simulink model "snap_adc5g_spec_rpi"  (R2019a)
settings: Solver=VariableStepDiscrete  StartTime=0.0  StopTime=10.0  RelTol=1e-3
undefined symbols (not defined in the file): pfb_coeff_gen_calc
libraries: xbsIndex_r4 x13965, casper_library_misc x80, casper_library_delays x43, xps_library x5, xbsReplacements_r4 x2, casper_library_communications x1
(part 133 of 152)

== system snap_adc5g_spec_rpi/fft_wideband_real/fft_biplex_real_4x/biplex_core/fft_stage_11/butterfly_direct/twiddle/bus_convert/conv3 ==
  note: (ones_bit & 1) -> round-to-even
      | (ones_bit ^ 1) -> round-to-odd
      | (sign_bit & 1)-> round-to-zero
      | (sign_bit ^ 1) -> round-to-inf
      | (X ~| 1) -> round half down
      | (X | 1) -> round half up
  in : Inport
  Concat : xbsIndex_r4/Concat  num_inputs=2  dbl_ovrd=off  block_type=concat
      settings: block_version=10.1.3
  Constant : xbsIndex_r4/Constant  const=1  gui_display_data_type=Fixed-point  arith_type=Unsigned  n_bits=1  bin_pt=0  preci_type=Single  exp_width=8  frac_width=24  explicit_period=off  period=1  equ=P=C  opselect=C  inp2=PCIN>>17  opr=+  inp1=P  carry=CIN  dbl_ovrd=off  block_type=constant
  Reinterpret : xbsIndex_r4/Reinterpret  force_arith_type=on  arith_type=Unsigned  force_bin_pt=on  bin_pt=0  block_type=reinterpret
      settings: infoedit="Changes signal type without altering the binary representation.   You can changed the signal between signed and unsigned, and relocate the binary point.<P><P>Hardware notes: In hardware this block costs nothing.<P><P>Example:  Suppose the input is 6 bits wide, signed, with 2 fractional bits, and the output is forced to unsigned with 0 fractional bits.  Then an input of -2.0 (1110.00 in binary 2's complement) becomes an output of 56 (111000 in binary)."  block_version=10.1.3
  adder : xbsIndex_r4/AddSub  mode=Addition  use_carryin=off  use_carryout=off  en=off  latency=1  precision=User Defined  arith_type="Signed  (2's comp)"  n_bits=19  bin_pt=17  quantization=Truncate  overflow=Wrap  use_behavioral_HDL=off  hw_selection=Fabric  pipelined=on  use_rpm=on  dbl_ovrd=off  block_type=addsub
      settings: xl_area=[0, 0, 0, 0, 0, 0, 0]  block_version=10.1.3
  almost_half : xbsIndex_r4/Constant  const=131071  gui_display_data_type=Fixed-point  arith_type=Unsigned  n_bits=35  bin_pt=0  preci_type=Single  exp_width=8  frac_width=24  explicit_period=off  period=1  equ=P=C  opselect=C  inp2=PCIN>>17  opr=+  inp1=P  carry=CIN  dbl_ovrd=off  block_type=constant
  bit : xbsIndex_r4/Slice  nbits=1  boolean_output=off  mode=Lower Bit Location + Width  bit1=0  base1=MSB of Input  bit0=17  base0=LSB of Input  dbl_ovrd=off  block_type=slice
      settings: infoedit="Extracts a given range of bits from each input sample and presents it at the output.  The output type is ordinarily unsigned with binary point at zero, but can be Boolean when the slice is one bit wide.<P><P>Hardware notes: In hardware this block costs nothing."  block_version=10.1.3
  force1 : xbsIndex_r4/Reinterpret  force_arith_type=on  arith_type="Signed  (2's comp)"  force_bin_pt=on  bin_pt=35  block_type=reinterpret
      settings: infoedit="Changes signal type without altering the binary representation.   You can changed the signal between signed and unsigned, and relocate the binary point.<P><P>Hardware notes: In hardware this block costs nothing.<P><P>Example:  Suppose the input is 6 bits wide, signed, with 2 fractional bits, and the output is forced to unsigned with 0 fractional bits.  Then an input of -2.0 (1110.00 in binary 2's complement) becomes an output of 56 (111000 in binary)."  block_version=10.1.3
  force2 : xbsIndex_r4/Reinterpret  force_arith_type=off  arith_type="Signed  (2's comp)"  force_bin_pt=on  bin_pt=35  block_type=reinterpret
      settings: infoedit="Changes signal type without altering the binary representation.   You can changed the signal between signed and unsigned, and relocate the binary point.<P><P>Hardware notes: In hardware this block costs nothing.<P><P>Example:  Suppose the input is 6 bits wide, signed, with 2 fractional bits, and the output is forced to unsigned with 0 fractional bits.  Then an input of -2.0 (1110.00 in binary 2's complement) becomes an output of 56 (111000 in binary)."  block_version=10.1.3
  tweak_op : xbsIndex_r4/Logical  logical_function=AND  inputs=2  en=off  latency=0  precision=Full  arith_type=Unsigned  n_bits=8  bin_pt=2  align_bp=on  dbl_ovrd=off  block_type=logical
      settings: xl_area=[0, 0, 0, 0, 0, 0, 0]
  out : Outport
  wires:
  tweak_op/1 -> Concat/2
  Constant/1 -> tweak_op/2
  bit/1 -> tweak_op/1
  almost_half/1 -> force2/1
  in/1 -> Reinterpret/1, bit/1
  Concat/1 -> force1/1
  Reinterpret/1 -> Concat/1
  force1/1 -> adder/1
  force2/1 -> adder/2
  adder/1 -> out/1

== system snap_adc5g_spec_rpi/fft_wideband_real/fft_biplex_real_4x/biplex_core/fft_stage_11/butterfly_direct/twiddle/bus_convert/conv4 ==
  note: (ones_bit & 1) -> round-to-even
      | (ones_bit ^ 1) -> round-to-odd
      | (sign_bit & 1)-> round-to-zero
      | (sign_bit ^ 1) -> round-to-inf
      | (X ~| 1) -> round half down
      | (X | 1) -> round half up
  in : Inport
  Concat : xbsIndex_r4/Concat  num_inputs=2  dbl_ovrd=off  block_type=concat
      settings: block_version=10.1.3
  Constant : xbsIndex_r4/Constant  const=1  gui_display_data_type=Fixed-point  arith_type=Unsigned  n_bits=1  bin_pt=0  preci_type=Single  exp_width=8  frac_width=24  explicit_period=off  period=1  equ=P=C  opselect=C  inp2=PCIN>>17  opr=+  inp1=P  carry=CIN  dbl_ovrd=off  block_type=constant
  Reinterpret : xbsIndex_r4/Reinterpret  force_arith_type=on  arith_type=Unsigned  force_bin_pt=on  bin_pt=0  block_type=reinterpret
      settings: infoedit="Changes signal type without altering the binary representation.   You can changed the signal between signed and unsigned, and relocate the binary point.<P><P>Hardware notes: In hardware this block costs nothing.<P><P>Example:  Suppose the input is 6 bits wide, signed, with 2 fractional bits, and the output is forced to unsigned with 0 fractional bits.  Then an input of -2.0 (1110.00 in binary 2's complement) becomes an output of 56 (111000 in binary)."  block_version=10.1.3
  adder : xbsIndex_r4/AddSub  mode=Addition  use_carryin=off  use_carryout=off  en=off  latency=1  precision=User Defined  arith_type="Signed  (2's comp)"  n_bits=19  bin_pt=17  quantization=Truncate  overflow=Wrap  use_behavioral_HDL=off  hw_selection=Fabric  pipelined=on  use_rpm=on  dbl_ovrd=off  block_type=addsub
      settings: xl_area=[0, 0, 0, 0, 0, 0, 0]  block_version=10.1.3
  almost_half : xbsIndex_r4/Constant  const=131071  gui_display_data_type=Fixed-point  arith_type=Unsigned  n_bits=35  bin_pt=0  preci_type=Single  exp_width=8  frac_width=24  explicit_period=off  period=1  equ=P=C  opselect=C  inp2=PCIN>>17  opr=+  inp1=P  carry=CIN  dbl_ovrd=off  block_type=constant
  bit : xbsIndex_r4/Slice  nbits=1  boolean_output=off  mode=Lower Bit Location + Width  bit1=0  base1=MSB of Input  bit0=17  base0=LSB of Input  dbl_ovrd=off  block_type=slice
      settings: infoedit="Extracts a given range of bits from each input sample and presents it at the output.  The output type is ordinarily unsigned with binary point at zero, but can be Boolean when the slice is one bit wide.<P><P>Hardware notes: In hardware this block costs nothing."  block_version=10.1.3
  force1 : xbsIndex_r4/Reinterpret  force_arith_type=on  arith_type="Signed  (2's comp)"  force_bin_pt=on  bin_pt=35  block_type=reinterpret
      settings: infoedit="Changes signal type without altering the binary representation.   You can changed the signal between signed and unsigned, and relocate the binary point.<P><P>Hardware notes: In hardware this block costs nothing.<P><P>Example:  Suppose the input is 6 bits wide, signed, with 2 fractional bits, and the output is forced to unsigned with 0 fractional bits.  Then an input of -2.0 (1110.00 in binary 2's complement) becomes an output of 56 (111000 in binary)."  block_version=10.1.3
  force2 : xbsIndex_r4/Reinterpret  force_arith_type=off  arith_type="Signed  (2's comp)"  force_bin_pt=on  bin_pt=35  block_type=reinterpret
      settings: infoedit="Changes signal type without altering the binary representation.   You can changed the signal between signed and unsigned, and relocate the binary point.<P><P>Hardware notes: In hardware this block costs nothing.<P><P>Example:  Suppose the input is 6 bits wide, signed, with 2 fractional bits, and the output is forced to unsigned with 0 fractional bits.  Then an input of -2.0 (1110.00 in binary 2's complement) becomes an output of 56 (111000 in binary)."  block_version=10.1.3
  tweak_op : xbsIndex_r4/Logical  logical_function=AND  inputs=2  en=off  latency=0  precision=Full  arith_type=Unsigned  n_bits=8  bin_pt=2  align_bp=on  dbl_ovrd=off  block_type=logical
      settings: xl_area=[0, 0, 0, 0, 0, 0, 0]
  out : Outport
  wires:
  tweak_op/1 -> Concat/2
  Constant/1 -> tweak_op/2
  bit/1 -> tweak_op/1
  almost_half/1 -> force2/1
  in/1 -> Reinterpret/1, bit/1
  Concat/1 -> force1/1
  Reinterpret/1 -> Concat/1
  force1/1 -> adder/1
  force2/1 -> adder/2
  adder/1 -> out/1

== system snap_adc5g_spec_rpi/fft_wideband_real/fft_biplex_real_4x/biplex_core/fft_stage_11/butterfly_direct/twiddle/bus_convert/debus ==
  bus_in : Inport
  reinterpret{1..4} (4 alike) : xbsIndex_r4/Reinterpret  force_arith_type=on  arith_type="Signed  (2's comp)"  force_bin_pt=on  bin_pt=34  block_type=reinterpret
  slice1 : xbsIndex_r4/Slice  nbits=37  boolean_output=off  mode=Upper Bit Location + Width  bit1=-111  base1=MSB of Input  bit0=0  base0=LSB of Input  dbl_ovrd=off  block_type=slice
  slice2 : xbsIndex_r4/Slice  nbits=37  boolean_output=off  mode=Upper Bit Location + Width  bit1=-74  base1=MSB of Input  bit0=0  base0=LSB of Input  dbl_ovrd=off  block_type=slice
  slice3 : xbsIndex_r4/Slice  nbits=37  boolean_output=off  mode=Upper Bit Location + Width  bit1=-37  base1=MSB of Input  bit0=0  base0=LSB of Input  dbl_ovrd=off  block_type=slice
  slice4 : xbsIndex_r4/Slice  nbits=37  boolean_output=off  mode=Upper Bit Location + Width  bit1=0  base1=MSB of Input  bit0=0  base0=LSB of Input  dbl_ovrd=off  block_type=slice
  msb_out4 : Outport
  out3 : Outport  Port=2
  out2 : Outport  Port=3
  lsb_out1 : Outport  Port=4
  wires:
  bus_in/1 -> slice4/1, slice3/1, slice2/1, slice1/1
  slice4/1 -> reinterpret4/1
  reinterpret4/1 -> msb_out4/1
  slice3/1 -> reinterpret3/1
  reinterpret3/1 -> out3/1
  slice2/1 -> reinterpret2/1
  reinterpret2/1 -> out2/1
  slice1/1 -> reinterpret1/1
  reinterpret1/1 -> lsb_out1/1

== system snap_adc5g_spec_rpi/fft_wideband_real/fft_biplex_real_4x/biplex_core/fft_stage_11/butterfly_direct/twiddle/bus_mult/a*b_bussify ==
  in1 : Inport
  in2 : Inport  Port=2
  concatenate : xbsIndex_r4/Concat  num_inputs=2  dbl_ovrd=off  block_type=concat
  reinterpret1 : xbsIndex_r4/Reinterpret  force_arith_type=on  arith_type=Unsigned  force_bin_pt=on  bin_pt=0  block_type=reinterpret
      settings: infoedit="Changes signal type without altering the binary representation.   You can changed the signal between signed and unsigned, and relocate the binary point.<br><br>Hardware notes: In hardware this block costs nothing.<br><br>Example:  Suppose the input is 6 bits wide, signed, with 2 fractional bits, and the output is forced to unsigned with 0 fractional bits.  Then an input of -2.0 (1110.00 in binary 2's complement) becomes an output of 56 (111000 in binary)."
  reinterpret2 : xbsIndex_r4/Reinterpret  force_arith_type=on  arith_type=Unsigned  force_bin_pt=on  bin_pt=0  block_type=reinterpret
      settings: infoedit="Changes signal type without altering the binary representation.   You can changed the signal between signed and unsigned, and relocate the binary point.<br><br>Hardware notes: In hardware this block costs nothing.<br><br>Example:  Suppose the input is 6 bits wide, signed, with 2 fractional bits, and the output is forced to unsigned with 0 fractional bits.  Then an input of -2.0 (1110.00 in binary 2's complement) becomes an output of 56 (111000 in binary)."
  bus_out : Outport
  wires:
  concatenate/1 -> bus_out/1
  in1/1 -> reinterpret1/1
  reinterpret1/1 -> concatenate/1
  in2/1 -> reinterpret2/1
  reinterpret2/1 -> concatenate/2

== system snap_adc5g_spec_rpi/fft_wideband_real/fft_biplex_real_4x/biplex_core/fft_stage_11/butterfly_direct/twiddle/bus_mult/a_debus ==
  bus_in : Inport
  reinterpret1 : xbsIndex_r4/Reinterpret  force_arith_type=on  arith_type=Unsigned  force_bin_pt=on  bin_pt=0  block_type=reinterpret
  slice1 : xbsIndex_r4/Slice  nbits=36  boolean_output=off  mode=Upper Bit Location + Width  bit1=0  base1=MSB of Input  bit0=0  base0=LSB of Input  dbl_ovrd=off  block_type=slice
  msb_lsb_out1 : Outport
  wires:
  bus_in/1 -> slice1/1
  slice1/1 -> reinterpret1/1
  reinterpret1/1 -> msb_lsb_out1/1

== system snap_adc5g_spec_rpi/fft_wideband_real/fft_biplex_real_4x/biplex_core/fft_stage_11/butterfly_direct/twiddle/bus_mult/b_debus ==
  bus_in : Inport
  reinterpret1 : xbsIndex_r4/Reinterpret  force_arith_type=on  arith_type=Unsigned  force_bin_pt=on  bin_pt=0  block_type=reinterpret
  reinterpret2 : xbsIndex_r4/Reinterpret  force_arith_type=on  arith_type=Unsigned  force_bin_pt=on  bin_pt=0  block_type=reinterpret
  slice1 : xbsIndex_r4/Slice  nbits=36  boolean_output=off  mode=Upper Bit Location + Width  bit1=-36  base1=MSB of Input  bit0=0  base0=LSB of Input  dbl_ovrd=off  block_type=slice
  slice2 : xbsIndex_r4/Slice  nbits=36  boolean_output=off  mode=Upper Bit Location + Width  bit1=0  base1=MSB of Input  bit0=0  base0=LSB of Input  dbl_ovrd=off  block_type=slice
  msb_out2 : Outport
  lsb_out1 : Outport  Port=2
  wires:
  bus_in/1 -> slice2/1, slice1/1
  slice2/1 -> reinterpret2/1
  reinterpret2/1 -> msb_out2/1
  slice1/1 -> reinterpret1/1
  reinterpret1/1 -> lsb_out1/1

== system snap_adc5g_spec_rpi/fft_wideband_real/fft_biplex_real_4x/biplex_core/fft_stage_11/butterfly_direct/twiddle/bus_mult/mult1 ==
  a : Inport
  b : Inport  Port=2
  a_expand : Subsystem  AncestorBlock=casper_library_flow_control/bus_expand  mask(bus_expand){mode=divisions of equal size, outputNum=4, outputWidth=[18 18 18 18], outputBinaryPt=[17 17 17 17], outputArithmeticType=[1 1 1 1], show_format=off, outputToWorkspace=off, variablePrefix=out, outputToModelAsWell=on}
      mask prompts: outputNum "Number of outputs:"; outputWidth "Output width:"; outputBinaryPt "Output binary point position:"; outputArithmeticType "Output arithmetic type (ufix=0, fix=1, bool=2):"; show_format "Print format string?"; outputToWorkspace "Output to workspace?"; variablePrefix "Variable name prefix:"; outputToModelAsWell "Output to model as well?"
      mask help:
      | Expands a 'bus' made using a bus_create or Xilinx
      | concat block.
      | The input will be divided into the specified number
      | of outputs with the specified arithmetic types.
      | Divisions are made from most significant bit.
      mask init: same as snap_adc5g_spec_rpi/ss_adc/ctrl_split
      settings: AttributesFormatString=4 outputs
      mask TypeOptions mode: divisions of equal size | divisions of arbitrary size
      mask Callback mode: bus_expand_callback();
      mask Callback outputWidth: bus_expand_callback();
      mask Callback outputToWorkspace: bus_expand_callback();
  a_replicate : Subsystem  AncestorBlock=casper_library_bus/bus_replicate  mask(bus_replicate){replication=2, csp_latency=1, misc=off, implementation=core}
      mask prompts: replication "replication factor"; csp_latency "latency"; misc "misc support"; implementation "delay implementation"
      mask help: Output bus formed by replicating input bus a number of times
      mask init:
      | bus_replicate_init(gcb, ...
      |     'replication', replication, ...
      |     'csp_latency', csp_latency, ...
      |     'implementation', implementation, ...
      |     'misc', misc);
      mask TypeOptions implementation: core | behavioral
  addsub_im : xbsIndex_r4/AddSub  mode=Addition  use_carryin=off  use_carryout=off  en=off  latency=1  precision=Full  arith_type=Unsigned  n_bits=16  bin_pt=14  quantization=Truncate  overflow=Wrap  use_behavioral_HDL=on  hw_selection=Fabric  pipelined=on  use_rpm=on  dbl_ovrd=off  block_type=addsub
  addsub_re : xbsIndex_r4/AddSub  mode=Subtraction  use_carryin=off  use_carryout=off  en=off  latency=1  precision=Full  arith_type=Unsigned  n_bits=16  bin_pt=14  quantization=Truncate  overflow=Wrap  use_behavioral_HDL=on  hw_selection=Fabric  pipelined=on  use_rpm=on  dbl_ovrd=off  block_type=addsub
  b_expand : Subsystem  AncestorBlock=casper_library_flow_control/bus_expand  mask(bus_expand){mode=divisions of equal size, outputNum=4, outputWidth=[18 18 18 18], outputBinaryPt=[17 17 17 17], outputArithmeticType=[1 1 1 1], show_format=off, outputToWorkspace=off, variablePrefix=out, outputToModelAsWell=on}
      mask prompts: outputNum "Number of outputs:"; outputWidth "Output width:"; outputBinaryPt "Output binary point position:"; outputArithmeticType "Output arithmetic type (ufix=0, fix=1, bool=2):"; show_format "Print format string?"; outputToWorkspace "Output to workspace?"; variablePrefix "Variable name prefix:"; outputToModelAsWell "Output to model as well?"
      mask help:
      | Expands a 'bus' made using a bus_create or Xilinx
      | concat block.
      | The input will be divided into the specified number
      | of outputs with the specified arithmetic types.
      | Divisions are made from most significant bit.
      mask init: same as snap_adc5g_spec_rpi/ss_adc/ctrl_split
      settings: AttributesFormatString=4 outputs
      mask TypeOptions mode: divisions of equal size | divisions of arbitrary size
      mask Callback mode: bus_expand_callback();
      mask Callback outputWidth: bus_expand_callback();
      mask Callback outputToWorkspace: bus_expand_callback();
  b_replicate : Subsystem  AncestorBlock=casper_library_bus/bus_replicate  mask(bus_replicate){replication=2, csp_latency=1, misc=off, implementation=core}
      mask prompts: replication "replication factor"; csp_latency "latency"; misc "misc support"; implementation "delay implementation"
      mask help: Output bus formed by replicating input bus a number of times
      mask init:
      | bus_replicate_init(gcb, ...
      |     'replication', replication, ...
      |     'csp_latency', csp_latency, ...
      |     'implementation', implementation, ...
      |     'misc', misc);
      mask TypeOptions implementation: core | behavioral
  convert_im : xbsIndex_r4/Convert  gui_display_data_type=Fixed-point  arith_type="Signed  (2's comp)"  n_bits=37  bin_pt=34  float_type=Single  exp_bits=8  fraction_bits=24  quantization=Truncate  overflow=Wrap  en=off  latency=0  pipeline=on  dbl_ovrd=off  block_type=convert
  convert_re : xbsIndex_r4/Convert  gui_display_data_type=Fixed-point  arith_type="Signed  (2's comp)"  n_bits=37  bin_pt=34  float_type=Single  exp_bits=8  fraction_bits=24  quantization=Truncate  overflow=Wrap  en=off  latency=0  pipeline=on  dbl_ovrd=off  block_type=convert
  imim : xbsIndex_r4/Mult  precision=Full  arith_type="Signed  (2's comp)"  n_bits=16  bin_pt=14  quantization=Truncate  overflow=Wrap  en=off  latency=2  use_behavioral_HDL=on  opt=Speed  use_embedded=off  optimum_pipeline=off  pipeline=on  dbl_ovrd=off  use_rpm=on  placement_style=Triangular  block_type=mult
  imre : xbsIndex_r4/Mult  precision=Full  arith_type="Signed  (2's comp)"  n_bits=16  bin_pt=14  quantization=Truncate  overflow=Wrap  en=off  latency=2  use_behavioral_HDL=on  opt=Speed  use_embedded=off  optimum_pipeline=off  pipeline=on  dbl_ovrd=off  use_rpm=on  placement_style=Triangular  block_type=mult
  reim : xbsIndex_r4/Mult  precision=Full  arith_type="Signed  (2's comp)"  n_bits=16  bin_pt=14  quantization=Truncate  overflow=Wrap  en=off  latency=2  use_behavioral_HDL=on  opt=Speed  use_embedded=off  optimum_pipeline=off  pipeline=on  dbl_ovrd=off  use_rpm=on  placement_style=Triangular  block_type=mult
  rere : xbsIndex_r4/Mult  precision=Full  arith_type="Signed  (2's comp)"  n_bits=16  bin_pt=14  quantization=Truncate  overflow=Wrap  en=off  latency=2  use_behavioral_HDL=on  opt=Speed  use_embedded=off  optimum_pipeline=off  pipeline=on  dbl_ovrd=off  use_rpm=on  placement_style=Triangular  block_type=mult
  ri_to_c : Subsystem  AncestorBlock=casper_library_misc/ri_to_c  mask(ri_to_c){}
      mask help:
      | Concatenates real and imaginary inputs into a complex output.
      | Useful for simplifying interconnects.
      | See also: Complex to Real-Imag (c_to_ri)
      mask Help: eval('xlWeb(''http://casper.berkeley.edu/wiki/Ri_to_c'')')
  ab : Outport
  wires:
  a/1 -> a_replicate/1(in)
  b/1 -> b_replicate/1(in)
  a_replicate/1(out) -> a_expand/1(bus_in)
  b_replicate/1(out) -> b_expand/1(bus_in)
  a_expand/1(msb_out4) -> rere/1
  b_expand/1(msb_out4) -> rere/2
  a_expand/2(out3) -> imim/1
  b_expand/2(out3) -> imim/2
  a_expand/4(lsb_out1) -> imre/1
  b_expand/3(out2) -> imre/2
  a_expand/3(out2) -> reim/1
  b_expand/4(lsb_out1) -> reim/2
  rere/1 -> addsub_re/1
  imim/1 -> addsub_re/2
  imre/1 -> addsub_im/1
  reim/1 -> addsub_im/2
  addsub_re/1 -> convert_re/1
  addsub_im/1 -> convert_im/1
  convert_re/1 -> ri_to_c/1(re)
  convert_im/1 -> ri_to_c/2(im)
  ri_to_c/1(c) -> ab/1

== system snap_adc5g_spec_rpi/fft_wideband_real/fft_biplex_real_4x/biplex_core/fft_stage_11/butterfly_direct/twiddle/bus_mult/mult2 ==
  a : Inport
  b : Inport  Port=2
  a_expand : Subsystem  AncestorBlock=casper_library_flow_control/bus_expand  mask(bus_expand){mode=divisions of equal size, outputNum=4, outputWidth=[18 18 18 18], outputBinaryPt=[17 17 17 17], outputArithmeticType=[1 1 1 1], show_format=off, outputToWorkspace=off, variablePrefix=out, outputToModelAsWell=on}
      mask prompts: outputNum "Number of outputs:"; outputWidth "Output width:"; outputBinaryPt "Output binary point position:"; outputArithmeticType "Output arithmetic type (ufix=0, fix=1, bool=2):"; show_format "Print format string?"; outputToWorkspace "Output to workspace?"; variablePrefix "Variable name prefix:"; outputToModelAsWell "Output to model as well?"
      mask help:
      | Expands a 'bus' made using a bus_create or Xilinx
      | concat block.
      | The input will be divided into the specified number
      | of outputs with the specified arithmetic types.
      | Divisions are made from most significant bit.
      mask init: same as snap_adc5g_spec_rpi/ss_adc/ctrl_split
      settings: AttributesFormatString=4 outputs
      mask TypeOptions mode: divisions of equal size | divisions of arbitrary size
      mask Callback mode: bus_expand_callback();
      mask Callback outputWidth: bus_expand_callback();
      mask Callback outputToWorkspace: bus_expand_callback();
  a_replicate : Subsystem  AncestorBlock=casper_library_bus/bus_replicate  mask(bus_replicate){replication=2, csp_latency=1, misc=off, implementation=core}
      mask prompts: replication "replication factor"; csp_latency "latency"; misc "misc support"; implementation "delay implementation"
      mask help: Output bus formed by replicating input bus a number of times
      mask init:
      | bus_replicate_init(gcb, ...
      |     'replication', replication, ...
      |     'csp_latency', csp_latency, ...
      |     'implementation', implementation, ...
      |     'misc', misc);
      mask TypeOptions implementation: core | behavioral
  addsub_im : xbsIndex_r4/AddSub  mode=Addition  use_carryin=off  use_carryout=off  en=off  latency=1  precision=Full  arith_type=Unsigned  n_bits=16  bin_pt=14  quantization=Truncate  overflow=Wrap  use_behavioral_HDL=on  hw_selection=Fabric  pipelined=on  use_rpm=on  dbl_ovrd=off  block_type=addsub
  addsub_re : xbsIndex_r4/AddSub  mode=Subtraction  use_carryin=off  use_carryout=off  en=off  latency=1  precision=Full  arith_type=Unsigned  n_bits=16  bin_pt=14  quantization=Truncate  overflow=Wrap  use_behavioral_HDL=on  hw_selection=Fabric  pipelined=on  use_rpm=on  dbl_ovrd=off  block_type=addsub
  b_expand : Subsystem  AncestorBlock=casper_library_flow_control/bus_expand  mask(bus_expand){mode=divisions of equal size, outputNum=4, outputWidth=[18 18 18 18], outputBinaryPt=[17 17 17 17], outputArithmeticType=[1 1 1 1], show_format=off, outputToWorkspace=off, variablePrefix=out, outputToModelAsWell=on}
      mask prompts: outputNum "Number of outputs:"; outputWidth "Output width:"; outputBinaryPt "Output binary point position:"; outputArithmeticType "Output arithmetic type (ufix=0, fix=1, bool=2):"; show_format "Print format string?"; outputToWorkspace "Output to workspace?"; variablePrefix "Variable name prefix:"; outputToModelAsWell "Output to model as well?"
      mask help:
      | Expands a 'bus' made using a bus_create or Xilinx
      | concat block.
      | The input will be divided into the specified number
      | of outputs with the specified arithmetic types.
      | Divisions are made from most significant bit.
      mask init: same as snap_adc5g_spec_rpi/ss_adc/ctrl_split
      settings: AttributesFormatString=4 outputs
      mask TypeOptions mode: divisions of equal size | divisions of arbitrary size
      mask Callback mode: bus_expand_callback();
      mask Callback outputWidth: bus_expand_callback();
      mask Callback outputToWorkspace: bus_expand_callback();
  b_replicate : Subsystem  AncestorBlock=casper_library_bus/bus_replicate  mask(bus_replicate){replication=2, csp_latency=1, misc=off, implementation=core}
      mask prompts: replication "replication factor"; csp_latency "latency"; misc "misc support"; implementation "delay implementation"
      mask help: Output bus formed by replicating input bus a number of times
      mask init:
      | bus_replicate_init(gcb, ...
      |     'replication', replication, ...
      |     'csp_latency', csp_latency, ...
      |     'implementation', implementation, ...
      |     'misc', misc);
      mask TypeOptions implementation: core | behavioral
  convert_im : xbsIndex_r4/Convert  gui_display_data_type=Fixed-point  arith_type="Signed  (2's comp)"  n_bits=37  bin_pt=34  float_type=Single  exp_bits=8  fraction_bits=24  quantization=Truncate  overflow=Wrap  en=off  latency=0  pipeline=on  dbl_ovrd=off  block_type=convert
  convert_re : xbsIndex_r4/Convert  gui_display_data_type=Fixed-point  arith_type="Signed  (2's comp)"  n_bits=37  bin_pt=34  float_type=Single  exp_bits=8  fraction_bits=24  quantization=Truncate  overflow=Wrap  en=off  latency=0  pipeline=on  dbl_ovrd=off  block_type=convert
  imim : xbsIndex_r4/Mult  precision=Full  arith_type="Signed  (2's comp)"  n_bits=16  bin_pt=14  quantization=Truncate  overflow=Wrap  en=off  latency=2  use_behavioral_HDL=on  opt=Speed  use_embedded=off  optimum_pipeline=off  pipeline=on  dbl_ovrd=off  use_rpm=on  placement_style=Triangular  block_type=mult
  imre : xbsIndex_r4/Mult  precision=Full  arith_type="Signed  (2's comp)"  n_bits=16  bin_pt=14  quantization=Truncate  overflow=Wrap  en=off  latency=2  use_behavioral_HDL=on  opt=Speed  use_embedded=off  optimum_pipeline=off  pipeline=on  dbl_ovrd=off  use_rpm=on  placement_style=Triangular  block_type=mult
  reim : xbsIndex_r4/Mult  precision=Full  arith_type="Signed  (2's comp)"  n_bits=16  bin_pt=14  quantization=Truncate  overflow=Wrap  en=off  latency=2  use_behavioral_HDL=on  opt=Speed  use_embedded=off  optimum_pipeline=off  pipeline=on  dbl_ovrd=off  use_rpm=on  placement_style=Triangular  block_type=mult
  rere : xbsIndex_r4/Mult  precision=Full  arith_type="Signed  (2's comp)"  n_bits=16  bin_pt=14  quantization=Truncate  overflow=Wrap  en=off  latency=2  use_behavioral_HDL=on  opt=Speed  use_embedded=off  optimum_pipeline=off  pipeline=on  dbl_ovrd=off  use_rpm=on  placement_style=Triangular  block_type=mult
  ri_to_c : Subsystem  AncestorBlock=casper_library_misc/ri_to_c  mask(ri_to_c){}
      mask help:
      | Concatenates real and imaginary inputs into a complex output.
      | Useful for simplifying interconnects.
      | See also: Complex to Real-Imag (c_to_ri)
      mask Help: eval('xlWeb(''http://casper.berkeley.edu/wiki/Ri_to_c'')')
  ab : Outport
  wires:
  a/1 -> a_replicate/1(in)
  b/1 -> b_replicate/1(in)
  a_replicate/1(out) -> a_expand/1(bus_in)
  b_replicate/1(out) -> b_expand/1(bus_in)
  a_expand/1(msb_out4) -> rere/1
  b_expand/1(msb_out4) -> rere/2
  a_expand/2(out3) -> imim/1
  b_expand/2(out3) -> imim/2
  a_expand/4(lsb_out1) -> imre/1
  b_expand/3(out2) -> imre/2
  a_expand/3(out2) -> reim/1
  b_expand/4(lsb_out1) -> reim/2
  rere/1 -> addsub_re/1
  imim/1 -> addsub_re/2
  imre/1 -> addsub_im/1
  reim/1 -> addsub_im/2
  addsub_re/1 -> convert_re/1
  addsub_im/1 -> convert_im/1
  convert_re/1 -> ri_to_c/1(re)
  convert_im/1 -> ri_to_c/2(im)
  ri_to_c/1(c) -> ab/1

== system snap_adc5g_spec_rpi/fft_wideband_real/fft_biplex_real_4x/biplex_core/fft_stage_11/butterfly_direct/twiddle/bus_mult/repa ==
  in : Inport
  bussify : Subsystem  AncestorBlock=casper_library_flow_control/bus_create  mask(bus_create){inputNum=1}
      mask prompts: inputNum "Number of inputs:"
      mask init:
      | bus_create_init(gcb,...
      |     'inputNum', inputNum);
  din0_0 : xbsIndex_r4/Delay  rst=off  infoeditControl=Selection of Reset will increase slice count due to use of real FFs and instead of SRLs  en=off  latency=1  reg_retiming=off  dbl_ovrd=off  block_type=delay
  out : Outport
  wires:
  in/1 -> din0_0/1
  din0_0/1 -> bussify/1(in1)
  bussify/1(bus_out) -> out/1

== system snap_adc5g_spec_rpi/fft_wideband_real/fft_biplex_real_4x/biplex_core/fft_stage_11/butterfly_direct/twiddle/bus_mult/repb ==
  in : Inport
  bussify : Subsystem  AncestorBlock=casper_library_flow_control/bus_create  mask(bus_create){inputNum=1}
      mask prompts: inputNum "Number of inputs:"
      mask init:
      | bus_create_init(gcb,...
      |     'inputNum', inputNum);
  din0_0 : xbsIndex_r4/Delay  rst=off  infoeditControl=Selection of Reset will increase slice count due to use of real FFs and instead of SRLs  en=off  latency=1  reg_retiming=off  dbl_ovrd=off  block_type=delay
  out : Outport
  wires:
  in/1 -> din0_0/1
  din0_0/1 -> bussify/1(in1)
  bussify/1(bus_out) -> out/1

== system snap_adc5g_spec_rpi/fft_wideband_real/fft_biplex_real_4x/biplex_core/fft_stage_11/butterfly_direct/twiddle/coeff_gen/bit_reverse ==
  in : Inport
  bit0 : xbsIndex_r4/Slice  nbits=1  boolean_output=off  mode=Lower Bit Location + Width  bit1=0  base1=MSB of Input  bit0=0  base0=LSB of Input  dbl_ovrd=off  block_type=slice
  bit1 : xbsIndex_r4/Slice  nbits=1  boolean_output=off  mode=Lower Bit Location + Width  bit1=0  base1=MSB of Input  bit0=1  base0=LSB of Input  dbl_ovrd=off  block_type=slice
  bit2 : xbsIndex_r4/Slice  nbits=1  boolean_output=off  mode=Lower Bit Location + Width  bit1=0  base1=MSB of Input  bit0=2  base0=LSB of Input  dbl_ovrd=off  block_type=slice
  bit3 : xbsIndex_r4/Slice  nbits=1  boolean_output=off  mode=Lower Bit Location + Width  bit1=0  base1=MSB of Input  bit0=3  base0=LSB of Input  dbl_ovrd=off  block_type=slice
  bit4 : xbsIndex_r4/Slice  nbits=1  boolean_output=off  mode=Lower Bit Location + Width  bit1=0  base1=MSB of Input  bit0=4  base0=LSB of Input  dbl_ovrd=off  block_type=slice
  bit5 : xbsIndex_r4/Slice  nbits=1  boolean_output=off  mode=Lower Bit Location + Width  bit1=0  base1=MSB of Input  bit0=5  base0=LSB of Input  dbl_ovrd=off  block_type=slice
  bit6 : xbsIndex_r4/Slice  nbits=1  boolean_output=off  mode=Lower Bit Location + Width  bit1=0  base1=MSB of Input  bit0=6  base0=LSB of Input  dbl_ovrd=off  block_type=slice
  bit7 : xbsIndex_r4/Slice  nbits=1  boolean_output=off  mode=Lower Bit Location + Width  bit1=0  base1=MSB of Input  bit0=7  base0=LSB of Input  dbl_ovrd=off  block_type=slice
  bit8 : xbsIndex_r4/Slice  nbits=1  boolean_output=off  mode=Lower Bit Location + Width  bit1=0  base1=MSB of Input  bit0=8  base0=LSB of Input  dbl_ovrd=off  block_type=slice
  bit9 : xbsIndex_r4/Slice  nbits=1  boolean_output=off  mode=Lower Bit Location + Width  bit1=0  base1=MSB of Input  bit0=9  base0=LSB of Input  dbl_ovrd=off  block_type=slice
  concat : xbsIndex_r4/Concat  num_inputs=10  dbl_ovrd=off  block_type=concat
  out : Outport
  wires:
  in/1 -> bit9/1, bit8/1, bit7/1, bit6/1, bit5/1, bit4/1, bit3/1, bit2/1, bit1/1, bit0/1
  bit9/1 -> concat/10
  bit8/1 -> concat/9
  bit7/1 -> concat/8
  bit6/1 -> concat/7
  bit5/1 -> concat/6
  bit4/1 -> concat/5
  bit3/1 -> concat/4
  bit2/1 -> concat/3
  bit1/1 -> concat/2
  bit0/1 -> concat/1
  concat/1 -> out/1

== system snap_adc5g_spec_rpi/fft_wideband_real/fft_biplex_real_4x/biplex_core/fft_stage_11/butterfly_direct/twiddle/coeff_gen/cosin ==
  theta : Inport
  misci : Inport  Port=2
  Constant : xbsIndex_r4/Constant  const=0  gui_display_data_type=Fixed-point  arith_type=Signed (2's comp)  n_bits=n_bits  bin_pt=bin_pt  preci_type=Single  exp_width=8  frac_width=24  explicit_period=off  period=1  equ=P=C  opselect=C  inp2=PCIN>>17  opr=+  inp1=P  carry=CIN  dbl_ovrd=off  block_type=constant
  Constant1 : xbsIndex_r4/Constant  const=0  gui_display_data_type=Fixed-point  arith_type=Signed (2's comp)  n_bits=n_bits  bin_pt=bin_pt  preci_type=Single  exp_width=8  frac_width=24  explicit_period=off  period=1  equ=P=C  opselect=C  inp2=PCIN>>17  opr=+  inp1=P  carry=CIN  dbl_ovrd=off  block_type=constant
  Constant2 : xbsIndex_r4/Constant  const=0  gui_display_data_type=Fixed-point  arith_type=Boolean  n_bits=n_bits  bin_pt=bin_pt  preci_type=Single  exp_width=8  frac_width=24  explicit_period=off  period=1  equ=P=C  opselect=C  inp2=PCIN>>17  opr=+  inp1=P  carry=CIN  dbl_ovrd=off  block_type=constant
  Constant3 : xbsIndex_r4/Constant  const=0  gui_display_data_type=Fixed-point  arith_type=Boolean  n_bits=n_bits  bin_pt=bin_pt  preci_type=Single  exp_width=8  frac_width=24  explicit_period=off  period=1  equ=P=C  opselect=C  inp2=PCIN>>17  opr=+  inp1=P  carry=CIN  dbl_ovrd=off  block_type=constant
  Constant4 : xbsIndex_r4/Constant  const=0  gui_display_data_type=Fixed-point  arith_type=Unsigned  n_bits=1  bin_pt=0  preci_type=Single  exp_width=8  frac_width=24  explicit_period=on  period=1  equ=P=C  opselect=C  inp2=PCIN>>17  opr=+  inp1=P  carry=CIN  dbl_ovrd=off  block_type=constant
  Constant5 : xbsIndex_r4/Constant  const=0  gui_display_data_type=Fixed-point  arith_type=Unsigned  n_bits=1  bin_pt=0  preci_type=Single  exp_width=8  frac_width=24  explicit_period=on  period=1  equ=P=C  opselect=C  inp2=PCIN>>17  opr=+  inp1=P  carry=CIN  dbl_ovrd=off  block_type=constant
  Delay : xbsIndex_r4/Delay  rst=off  infoeditControl=Selection of Reset will increase slice count due to use of real FFs and instead of SRLs  en=off  latency=bram_latency  reg_retiming=on  dbl_ovrd=off  block_type=delay
  Delay10 : xbsIndex_r4/Delay  rst=off  infoeditControl=Selection of Reset will increase slice count due to use of real FFs and instead of SRLs  en=off  latency=bram_latency  reg_retiming=on  dbl_ovrd=off  block_type=delay
  Delay8 : xbsIndex_r4/Delay  rst=off  infoeditControl=Selection of Reset will increase slice count due to use of real FFs and instead of SRLs  en=off  latency=bram_latency  reg_retiming=on  dbl_ovrd=off  block_type=delay
  Terminator : Terminator
  Terminator1 : Terminator
  add_convert0 : Subsystem
  add_convert1 : Subsystem
  assert : xbsIndex_r4/Assert  assert_type=on  type_source=Explicitly  gui_display_data_type=Fixed-point  arith_type=Unsigned  n_bits=10  bin_pt=0  preci_type=Single  exp_width=8  frac_width=24  assert_rate=off  rate_source=Explicitly  period=1  output_port=on  block_type=assert
  invert0 : Subsystem  mask{n_bits=n_bits, bin_pt=bin_pt, neg_latency=neg_latency, mux_latency=mux_latency}
      mask prompts: n_bits "bit width"; bin_pt "binary point"; neg_latency "negate latency"; mux_latency "mux latency"
  invert1 : Subsystem  mask{n_bits=n_bits, bin_pt=bin_pt, neg_latency=neg_latency, mux_latency=mux_latency}
      mask prompts: n_bits "bit width"; bin_pt "binary point"; neg_latency "negate latency"; mux_latency "mux latency"
  lookup : xbsIndex_r4/Dual Port RAM  depth=2^(10)  initVector=cos((0*(2*pi))+(2*pi)/(2^11)*(0:(2^10)-1))  distributed_mem=Block RAM  init_a=0  init_b=0  rst_a=off  rst_b=off  en_a=off  en_b=off  latency=bram_latency  write_mode_A=Read After Write  write_mode_B=Read After Write  optimize=Area  dbl_ovrd=off  block_type=dpram
  cos : Outport
  -sin : Outport  Port=2
  misco : Outport  Port=3
  wires:
  theta/1 -> assert/1
  assert/1 -> add_convert0/1(theta), add_convert1/1(theta)
  Constant4/1 -> add_convert0/2(misci)
  add_convert0/3(misco) -> Terminator/1
  misci/1 -> add_convert1/2(misci)
  add_convert1/3(misco) -> Delay/1
  add_convert0/2(add) -> lookup/1
  add_convert1/2(add) -> lookup/4
  Constant/1 -> lookup/2
  Constant2/1 -> lookup/3
  Constant1/1 -> lookup/5
  Constant3/1 -> lookup/6
  add_convert1/1(negate) -> Delay8/1
  add_convert0/1(negate) -> Delay10/1
  Delay10/1 -> invert0/1(negate)
  Constant5/1 -> invert0/3(misci)
  lookup/1 -> invert0/2(in)
  Delay8/1 -> invert1/1(negate)
  lookup/2 -> invert1/2(in)
  invert0/2(misco) -> Terminator1/1
  Delay/1 -> invert1/3(misci)
  invert0/1(out) -> cos/1
  invert1/1(out) -> -sin/1
  invert1/2(misco) -> misco/1

== system snap_adc5g_spec_rpi/fft_wideband_real/fft_biplex_real_4x/biplex_core/fft_stage_2/butterfly_direct/bus_convert/conv1/convert ==
  note: (ones_bit & 1) -> round-to-even
      | (ones_bit ^ 1) -> round-to-odd
      | (sign_bit & 1)-> round-to-zero
      | (sign_bit ^ 1) -> round-to-inf
      | (X ~| 1) -> round half down
      | (X | 1) -> round half up
  in : Inport
  Concat : xbsIndex_r4/Concat  num_inputs=2  dbl_ovrd=off  block_type=concat
      settings: block_version=10.1.3
  Constant : xbsIndex_r4/Constant  const=1  gui_display_data_type=Fixed-point  arith_type=Unsigned  n_bits=1  bin_pt=0  preci_type=Single  exp_width=8  frac_width=24  explicit_period=off  period=1  equ=P=C  opselect=C  inp2=PCIN>>17  opr=+  inp1=P  carry=CIN  dbl_ovrd=off  block_type=constant
  Reinterpret : xbsIndex_r4/Reinterpret  force_arith_type=on  arith_type=Unsigned  force_bin_pt=on  bin_pt=0  block_type=reinterpret
      settings: infoedit="Changes signal type without altering the binary representation.   You can changed the signal between signed and unsigned, and relocate the binary point.<P><P>Hardware notes: In hardware this block costs nothing.<P><P>Example:  Suppose the input is 6 bits wide, signed, with 2 fractional bits, and the output is forced to unsigned with 0 fractional bits.  Then an input of -2.0 (1110.00 in binary 2's complement) becomes an output of 56 (111000 in binary)."  block_version=10.1.3
  adder : xbsIndex_r4/AddSub  mode=Addition  use_carryin=off  use_carryout=off  en=off  latency=1  precision=User Defined  arith_type="Signed  (2's comp)"  n_bits=18  bin_pt=17  quantization=Truncate  overflow=Wrap  use_behavioral_HDL=off  hw_selection=Fabric  pipelined=on  use_rpm=on  dbl_ovrd=off  block_type=addsub
      settings: xl_area=[0, 0, 0, 0, 0, 0, 0]  block_version=10.1.3
  almost_half : xbsIndex_r4/Constant  const=1  gui_display_data_type=Fixed-point  arith_type=Unsigned  n_bits=19  bin_pt=0  preci_type=Single  exp_width=8  frac_width=24  explicit_period=off  period=1  equ=P=C  opselect=C  inp2=PCIN>>17  opr=+  inp1=P  carry=CIN  dbl_ovrd=off  block_type=constant
  bit : xbsIndex_r4/Slice  nbits=1  boolean_output=off  mode=Lower Bit Location + Width  bit1=0  base1=MSB of Input  bit0=1  base0=LSB of Input  dbl_ovrd=off  block_type=slice
      settings: infoedit="Extracts a given range of bits from each input sample and presents it at the output.  The output type is ordinarily unsigned with binary point at zero, but can be Boolean when the slice is one bit wide.<P><P>Hardware notes: In hardware this block costs nothing."  block_version=10.1.3
  force1 : xbsIndex_r4/Reinterpret  force_arith_type=on  arith_type="Signed  (2's comp)"  force_bin_pt=on  bin_pt=19  block_type=reinterpret
      settings: infoedit="Changes signal type without altering the binary representation.   You can changed the signal between signed and unsigned, and relocate the binary point.<P><P>Hardware notes: In hardware this block costs nothing.<P><P>Example:  Suppose the input is 6 bits wide, signed, with 2 fractional bits, and the output is forced to unsigned with 0 fractional bits.  Then an input of -2.0 (1110.00 in binary 2's complement) becomes an output of 56 (111000 in binary)."  block_version=10.1.3
  force2 : xbsIndex_r4/Reinterpret  force_arith_type=off  arith_type="Signed  (2's comp)"  force_bin_pt=on  bin_pt=19  block_type=reinterpret
      settings: infoedit="Changes signal type without altering the binary representation.   You can changed the signal between signed and unsigned, and relocate the binary point.<P><P>Hardware notes: In hardware this block costs nothing.<P><P>Example:  Suppose the input is 6 bits wide, signed, with 2 fractional bits, and the output is forced to unsigned with 0 fractional bits.  Then an input of -2.0 (1110.00 in binary 2's complement) becomes an output of 56 (111000 in binary)."  block_version=10.1.3
  tweak_op : xbsIndex_r4/Logical  logical_function=AND  inputs=2  en=off  latency=0  precision=Full  arith_type=Unsigned  n_bits=8  bin_pt=2  align_bp=on  dbl_ovrd=off  block_type=logical
      settings: xl_area=[0, 0, 0, 0, 0, 0, 0]
  out : Outport
  wires:
  tweak_op/1 -> Concat/2
  Constant/1 -> tweak_op/2
  bit/1 -> tweak_op/1
  almost_half/1 -> force2/1
  in/1 -> Reinterpret/1, bit/1
  Concat/1 -> force1/1
  Reinterpret/1 -> Concat/1
  force1/1 -> adder/1
  force2/1 -> adder/2
  adder/1 -> out/1

== system snap_adc5g_spec_rpi/fft_wideband_real/fft_biplex_real_4x/biplex_core/fft_stage_2/butterfly_direct/bus_convert/conv2/convert ==
  note: (ones_bit & 1) -> round-to-even
      | (ones_bit ^ 1) -> round-to-odd
      | (sign_bit & 1)-> round-to-zero
      | (sign_bit ^ 1) -> round-to-inf
      | (X ~| 1) -> round half down
      | (X | 1) -> round half up
  in : Inport
  Concat : xbsIndex_r4/Concat  num_inputs=2  dbl_ovrd=off  block_type=concat
      settings: block_version=10.1.3
  Constant : xbsIndex_r4/Constant  const=1  gui_display_data_type=Fixed-point  arith_type=Unsigned  n_bits=1  bin_pt=0  preci_type=Single  exp_width=8  frac_width=24  explicit_period=off  period=1  equ=P=C  opselect=C  inp2=PCIN>>17  opr=+  inp1=P  carry=CIN  dbl_ovrd=off  block_type=constant
  Reinterpret : xbsIndex_r4/Reinterpret  force_arith_type=on  arith_type=Unsigned  force_bin_pt=on  bin_pt=0  block_type=reinterpret
      settings: infoedit="Changes signal type without altering the binary representation.   You can changed the signal between signed and unsigned, and relocate the binary point.<P><P>Hardware notes: In hardware this block costs nothing.<P><P>Example:  Suppose the input is 6 bits wide, signed, with 2 fractional bits, and the output is forced to unsigned with 0 fractional bits.  Then an input of -2.0 (1110.00 in binary 2's complement) becomes an output of 56 (111000 in binary)."  block_version=10.1.3
  adder : xbsIndex_r4/AddSub  mode=Addition  use_carryin=off  use_carryout=off  en=off  latency=1  precision=User Defined  arith_type="Signed  (2's comp)"  n_bits=18  bin_pt=17  quantization=Truncate  overflow=Wrap  use_behavioral_HDL=off  hw_selection=Fabric  pipelined=on  use_rpm=on  dbl_ovrd=off  block_type=addsub
      settings: xl_area=[0, 0, 0, 0, 0, 0, 0]  block_version=10.1.3
  almost_half : xbsIndex_r4/Constant  const=1  gui_display_data_type=Fixed-point  arith_type=Unsigned  n_bits=19  bin_pt=0  preci_type=Single  exp_width=8  frac_width=24  explicit_period=off  period=1  equ=P=C  opselect=C  inp2=PCIN>>17  opr=+  inp1=P  carry=CIN  dbl_ovrd=off  block_type=constant
  bit : xbsIndex_r4/Slice  nbits=1  boolean_output=off  mode=Lower Bit Location + Width  bit1=0  base1=MSB of Input  bit0=1  base0=LSB of Input  dbl_ovrd=off  block_type=slice
      settings: infoedit="Extracts a given range of bits from each input sample and presents it at the output.  The output type is ordinarily unsigned with binary point at zero, but can be Boolean when the slice is one bit wide.<P><P>Hardware notes: In hardware this block costs nothing."  block_version=10.1.3
  force1 : xbsIndex_r4/Reinterpret  force_arith_type=on  arith_type="Signed  (2's comp)"  force_bin_pt=on  bin_pt=19  block_type=reinterpret
      settings: infoedit="Changes signal type without altering the binary representation.   You can changed the signal between signed and unsigned, and relocate the binary point.<P><P>Hardware notes: In hardware this block costs nothing.<P><P>Example:  Suppose the input is 6 bits wide, signed, with 2 fractional bits, and the output is forced to unsigned with 0 fractional bits.  Then an input of -2.0 (1110.00 in binary 2's complement) becomes an output of 56 (111000 in binary)."  block_version=10.1.3
  force2 : xbsIndex_r4/Reinterpret  force_arith_type=off  arith_type="Signed  (2's comp)"  force_bin_pt=on  bin_pt=19  block_type=reinterpret
      settings: infoedit="Changes signal type without altering the binary representation.   You can changed the signal between signed and unsigned, and relocate the binary point.<P><P>Hardware notes: In hardware this block costs nothing.<P><P>Example:  Suppose the input is 6 bits wide, signed, with 2 fractional bits, and the output is forced to unsigned with 0 fractional bits.  Then an input of -2.0 (1110.00 in binary 2's complement) becomes an output of 56 (111000 in binary)."  block_version=10.1.3
  tweak_op : xbsIndex_r4/Logical  logical_function=AND  inputs=2  en=off  latency=0  precision=Full  arith_type=Unsigned  n_bits=8  bin_pt=2  align_bp=on  dbl_ovrd=off  block_type=logical
      settings: xl_area=[0, 0, 0, 0, 0, 0, 0]
  out : Outport
  wires:
  tweak_op/1 -> Concat/2
  Constant/1 -> tweak_op/2
  bit/1 -> tweak_op/1
  almost_half/1 -> force2/1
  in/1 -> Reinterpret/1, bit/1
  Concat/1 -> force1/1
  Reinterpret/1 -> Concat/1
  force1/1 -> adder/1
  force2/1 -> adder/2
  adder/1 -> out/1
